simulink model "Vataleni_PMSG_SSO_Final"  (R2025b)
settings: Solver=ode4  StartTime=0.0  StopTime=12  FixedStep=0.00020000000000000001  RelTol=1e-3
model workspace (MAT data in the model file):
  grid_disturbance_time = 2
  mitigation_enable = 0
  scr_final = 10
  scr_initial = 10
  wind_nom = 12
  wind_step = 12
  wind_step_time = 4
settings Model: Creator=Tsenaye  LastModifiedBy=Tsenaye
settings DataIOCC: SignalLogging=off
settings DebuggingCC: AlgebraicLoopMsg=error  UnconnectedInputMsg=error  UnconnectedOutputMsg=warning  UnconnectedLineMsg=error

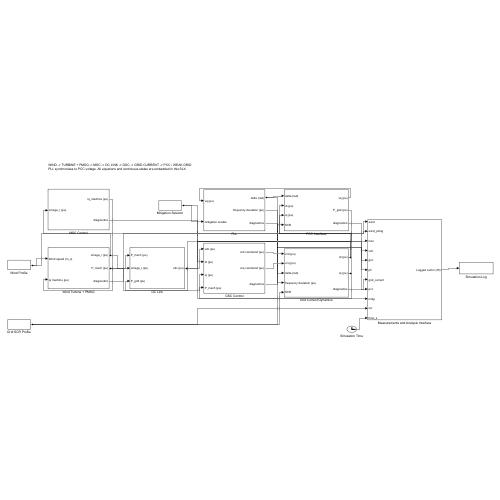
[thumbnail: Simulink's stored preview of the top-level diagram]
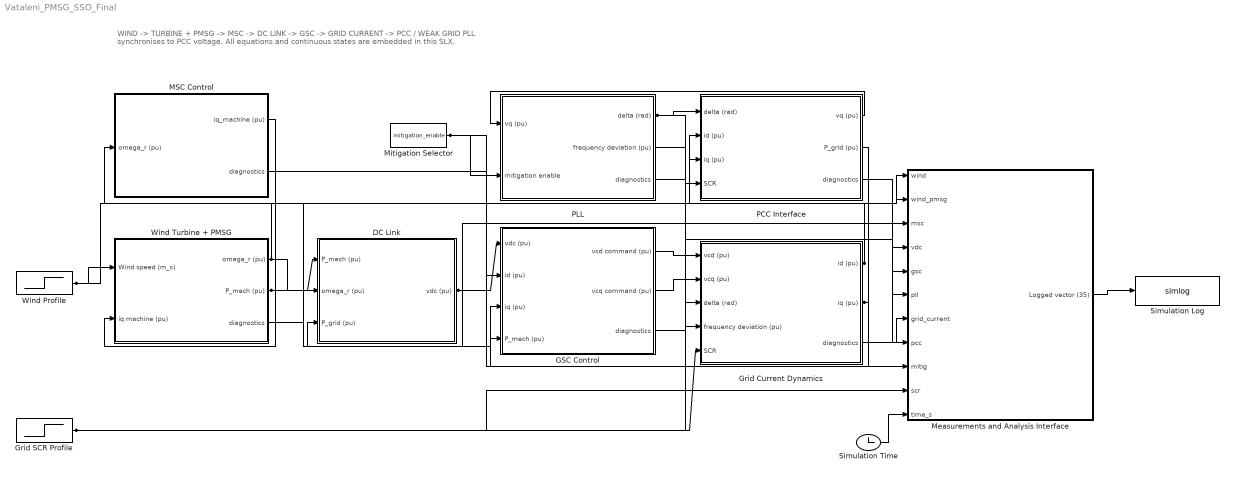
== system Vataleni_PMSG_SSO_Final ==
  note: WIND -> TURBINE + PMSG -> MSC -> DC LINK -> GSC -> GRID CURRENT -> PCC / WEAK GRID
      | PLL synchronises to PCC voltage. All equations and continuous states are embedded in this SLX.
  DC Link : Subsystem
  GSC Control : Subsystem
  Grid Current Dynamics : Subsystem
  Grid SCR Profile : Step  Time=grid_disturbance_time  Before=scr_initial  After=scr_final  SampleTime=0
  MSC Control : Subsystem
  Measurements and Analysis Interface : Subsystem
  Mitigation Selector : Constant  Value=mitigation_enable
  PCC Interface : Subsystem
  PLL : Subsystem
  Simulation Log : ToWorkspace  VariableName=simlog  SampleTime=-1
  Simulation Time : Clock
  Wind Profile : Step  Time=wind_step_time  Before=wind_nom  After=wind_step  SampleTime=0
  Wind Turbine + PMSG : Subsystem
  wires:
  Wind Profile/1 -> Wind Turbine + PMSG/1(Wind speed (m_s)), Measurements and Analysis Interface/1(wind)
  MSC Control/1(iq_machine (pu)) -> Wind Turbine + PMSG/2(iq machine (pu))
  Wind Turbine + PMSG/1(omega_r (pu)) -> MSC Control/1(omega_r (pu)), DC Link/2(omega_r (pu))
  Wind Turbine + PMSG/2(P_mech (pu)) -> DC Link/1(P_mech (pu)), GSC Control/4(P_mech (pu))
  PCC Interface/2(P_grid (pu)) -> DC Link/3(P_grid (pu))
  DC Link/1(vdc (pu)) -> GSC Control/1(vdc (pu)), Measurements and Analysis Interface/4(vdc)
  Grid Current Dynamics/1(id (pu)) -> GSC Control/2(id (pu)), PCC Interface/2(id (pu))
  Grid Current Dynamics/2(iq (pu)) -> GSC Control/3(iq (pu)), PCC Interface/3(iq (pu))
  PCC Interface/1(vq (pu)) -> PLL/1(vq (pu))
  Mitigation Selector/1 -> PLL/2(mitigation enable), Measurements and Analysis Interface/9(mitig)
  GSC Control/1(vcd command (pu)) -> Grid Current Dynamics/1(vcd (pu))
  GSC Control/2(vcq command (pu)) -> Grid Current Dynamics/2(vcq (pu))
  PLL/1(delta (rad)) -> Grid Current Dynamics/3(delta (rad)), PCC Interface/1(delta (rad))
  PLL/2(frequency deviation (pu)) -> Grid Current Dynamics/4(frequency deviation (pu))
  Grid SCR Profile/1 -> Grid Current Dynamics/5(SCR), PCC Interface/4(SCR), Measurements and Analysis Interface/10(scr)
  Wind Turbine + PMSG/3(diagnostics) -> Measurements and Analysis Interface/2(wind_pmsg)
  MSC Control/2(diagnostics) -> Measurements and Analysis Interface/3(msc)
  GSC Control/3(diagnostics) -> Measurements and Analysis Interface/5(gsc)
  PLL/3(diagnostics) -> Measurements and Analysis Interface/6(pll)
  Grid Current Dynamics/3(diagnostics) -> Measurements and Analysis Interface/7(grid_current)
  PCC Interface/3(diagnostics) -> Measurements and Analysis Interface/8(pcc)
  Simulation Time/1 -> Measurements and Analysis Interface/11(time_s)
  Measurements and Analysis Interface/1(Logged vector (35)) -> Simulation Log/1

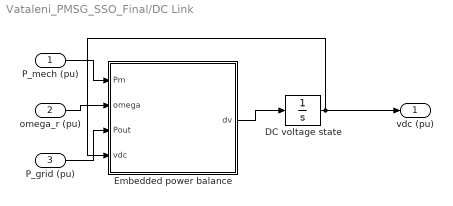
== system Vataleni_PMSG_SSO_Final/DC Link ==
  P_mech (pu) : Inport
  omega_r (pu) : Inport  Port=2
  P_grid (pu) : Inport  Port=3
  DC voltage state : Integrator  InitialCondition=1
  Embedded power balance : MATLAB Function  TreatAsAtomicUnit=on
  vdc (pu) : Outport
  wires:
  P_mech (pu)/1 -> Embedded power balance/1(Pm)
  omega_r (pu)/1 -> Embedded power balance/2(omega)
  P_grid (pu)/1 -> Embedded power balance/3(Pout)
  DC voltage state/1 -> Embedded power balance/4(vdc), vdc (pu)/1
  Embedded power balance/1(dv) -> DC voltage state/1

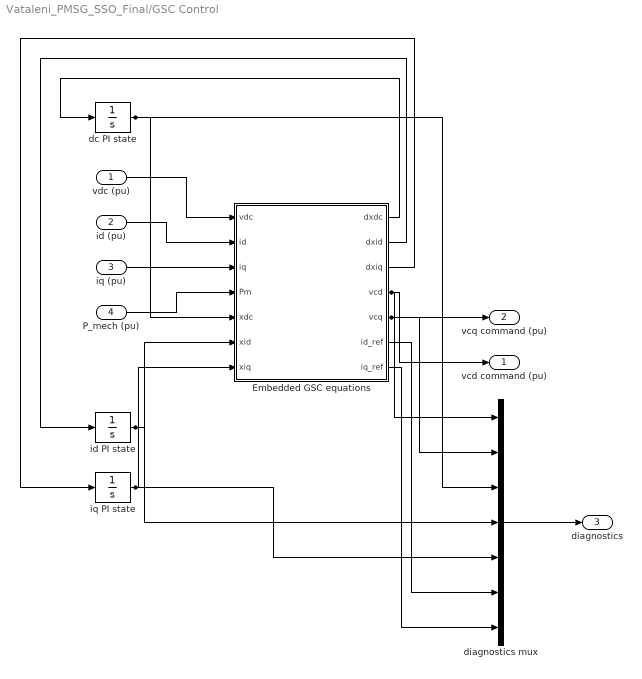
== system Vataleni_PMSG_SSO_Final/GSC Control ==
  vdc (pu) : Inport
  id (pu) : Inport  Port=2
  iq (pu) : Inport  Port=3
  P_mech (pu) : Inport  Port=4
  Embedded GSC equations : MATLAB Function  TreatAsAtomicUnit=on
  dc PI state : Integrator  InitialCondition=-0.0043132729709667306
  diagnostics mux : Mux  Inputs=7
  id PI state : Integrator  InitialCondition=0.013689040731538427
  iq PI state : Integrator
  vcd command (pu) : Outport
  vcq command (pu) : Outport  Port=2
  diagnostics : Outport  Port=3
  wires:
  vdc (pu)/1 -> Embedded GSC equations/1(vdc)
  iq PI state/1 -> diagnostics mux/5, Embedded GSC equations/7(xiq)
  Embedded GSC equations/1(dxdc) -> dc PI state/1
  id PI state/1 -> diagnostics mux/4, Embedded GSC equations/6(xid)
  dc PI state/1 -> diagnostics mux/3, Embedded GSC equations/5(xdc)
  P_mech (pu)/1 -> Embedded GSC equations/4(Pm)
  iq (pu)/1 -> Embedded GSC equations/3(iq)
  id (pu)/1 -> Embedded GSC equations/2(id)
  Embedded GSC equations/2(dxid) -> id PI state/1
  Embedded GSC equations/3(dxiq) -> iq PI state/1
  Embedded GSC equations/4(vcd) -> vcd command (pu)/1, diagnostics mux/1
  Embedded GSC equations/5(vcq) -> vcq command (pu)/1, diagnostics mux/2
  Embedded GSC equations/6(id_ref) -> diagnostics mux/6
  Embedded GSC equations/7(iq_ref) -> diagnostics mux/7
  diagnostics mux/1 -> diagnostics/1

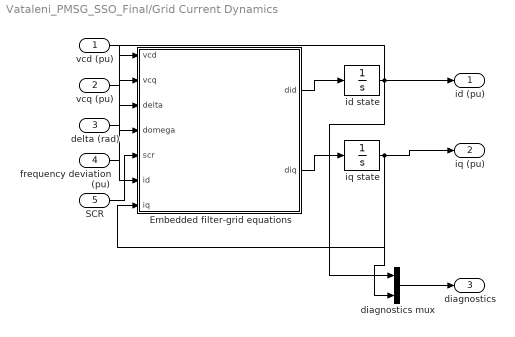
== system Vataleni_PMSG_SSO_Final/Grid Current Dynamics ==
  vcd (pu) : Inport
  vcq (pu) : Inport  Port=2
  delta (rad) : Inport  Port=3
  frequency deviation (pu) : Inport  Port=4
  SCR : Inport  Port=5
  Embedded filter-grid equations : MATLAB Function  TreatAsAtomicUnit=on
  diagnostics mux : Mux  Inputs=2
  id state : Integrator  InitialCondition=0.8771883675516966
  iq state : Integrator
  id (pu) : Outport
  iq (pu) : Outport  Port=2
  diagnostics : Outport  Port=3
  wires:
  vcd (pu)/1 -> Embedded filter-grid equations/1(vcd)
  vcq (pu)/1 -> Embedded filter-grid equations/2(vcq)
  delta (rad)/1 -> Embedded filter-grid equations/3(delta)
  frequency deviation (pu)/1 -> Embedded filter-grid equations/4(domega)
  SCR/1 -> Embedded filter-grid equations/5(scr)
  id state/1 -> Embedded filter-grid equations/6(id), id (pu)/1, diagnostics mux/1
  iq state/1 -> Embedded filter-grid equations/7(iq), iq (pu)/1, diagnostics mux/2
  Embedded filter-grid equations/1(did) -> id state/1
  Embedded filter-grid equations/2(diq) -> iq state/1
  diagnostics mux/1 -> diagnostics/1

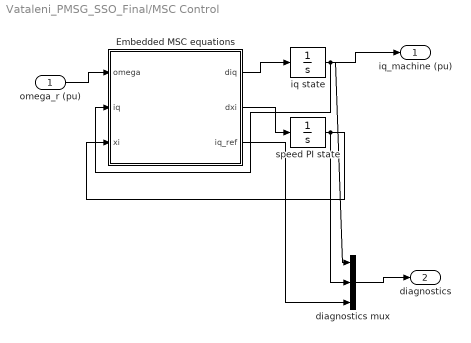
== system Vataleni_PMSG_SSO_Final/MSC Control ==
  omega_r (pu) : Inport
  Embedded MSC equations : MATLAB Function  TreatAsAtomicUnit=on
  diagnostics mux : Mux  Inputs=3
  iq state : Integrator  InitialCondition=0.88150164052266333
  speed PI state : Integrator  InitialCondition=0.88150164052266333
  iq_machine (pu) : Outport
  diagnostics : Outport  Port=2
  wires:
  omega_r (pu)/1 -> Embedded MSC equations/1(omega)
  iq state/1 -> Embedded MSC equations/2(iq), iq_machine (pu)/1, diagnostics mux/1
  speed PI state/1 -> Embedded MSC equations/3(xi), diagnostics mux/2
  Embedded MSC equations/1(diq) -> iq state/1
  Embedded MSC equations/2(dxi) -> speed PI state/1
  Embedded MSC equations/3(iq_ref) -> diagnostics mux/3
  diagnostics mux/1 -> diagnostics/1

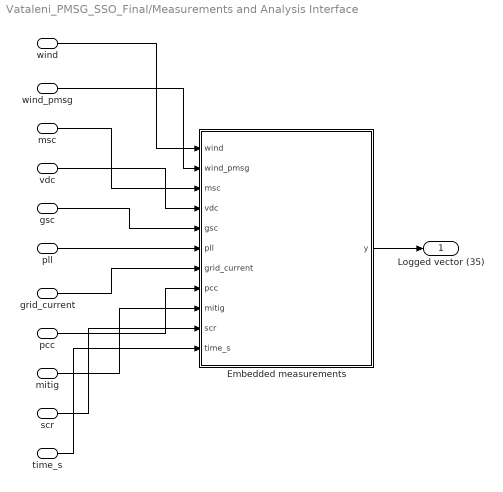
== system Vataleni_PMSG_SSO_Final/Measurements and Analysis Interface ==
  wind : Inport
  wind_pmsg : Inport  Port=2
  msc : Inport  Port=3
  vdc : Inport  Port=4
  gsc : Inport  Port=5
  pll : Inport  Port=6
  grid_current : Inport  Port=7
  pcc : Inport  Port=8
  mitig : Inport  Port=9
  scr : Inport  Port=10
  time_s : Inport  Port=11
  Embedded measurements : MATLAB Function  TreatAsAtomicUnit=on
  Logged vector (35) : Outport
  wires:
  grid_current/1 -> Embedded measurements/7(grid_current)
  gsc/1 -> Embedded measurements/5(gsc)
  time_s/1 -> Embedded measurements/11(time_s)
  msc/1 -> Embedded measurements/3(msc)
  wind/1 -> Embedded measurements/1(wind)
  pcc/1 -> Embedded measurements/8(pcc)
  Embedded measurements/1(y) -> Logged vector (35)/1
  pll/1 -> Embedded measurements/6(pll)
  vdc/1 -> Embedded measurements/4(vdc)
  scr/1 -> Embedded measurements/10(scr)
  wind_pmsg/1 -> Embedded measurements/2(wind_pmsg)
  mitig/1 -> Embedded measurements/9(mitig)

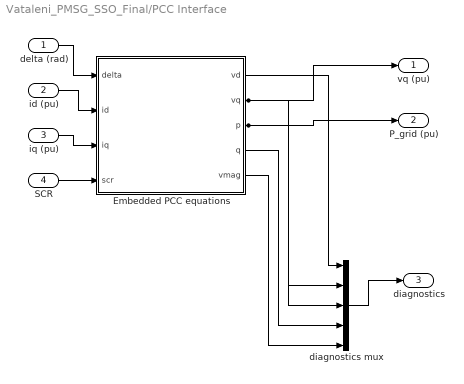
== system Vataleni_PMSG_SSO_Final/PCC Interface ==
  delta (rad) : Inport
  id (pu) : Inport  Port=2
  iq (pu) : Inport  Port=3
  SCR : Inport  Port=4
  Embedded PCC equations : MATLAB Function  TreatAsAtomicUnit=on
  diagnostics mux : Mux  Inputs=5
  vq (pu) : Outport
  P_grid (pu) : Outport  Port=2
  diagnostics : Outport  Port=3
  wires:
  delta (rad)/1 -> Embedded PCC equations/1(delta)
  id (pu)/1 -> Embedded PCC equations/2(id)
  iq (pu)/1 -> Embedded PCC equations/3(iq)
  SCR/1 -> Embedded PCC equations/4(scr)
  Embedded PCC equations/2(vq) -> vq (pu)/1, diagnostics mux/2
  Embedded PCC equations/3(p) -> P_grid (pu)/1, diagnostics mux/3
  Embedded PCC equations/1(vd) -> diagnostics mux/1
  Embedded PCC equations/4(q) -> diagnostics mux/4
  Embedded PCC equations/5(vmag) -> diagnostics mux/5
  diagnostics mux/1 -> diagnostics/1

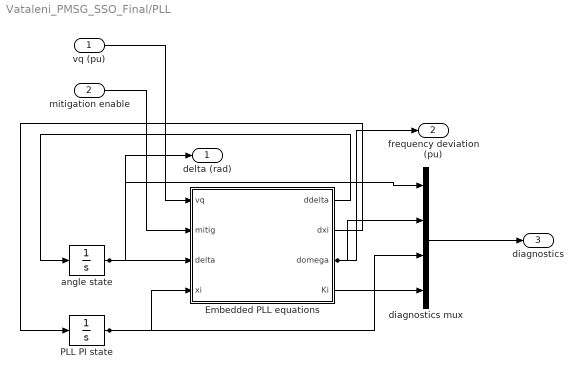
== system Vataleni_PMSG_SSO_Final/PLL ==
  vq (pu) : Inport
  mitigation enable : Inport  Port=2
  Embedded PLL equations : MATLAB Function  TreatAsAtomicUnit=on
  PLL PI state : Integrator
  angle state : Integrator  InitialCondition=0.087831721542046673
  diagnostics mux : Mux
  delta (rad) : Outport
  frequency deviation (pu) : Outport  Port=2
  diagnostics : Outport  Port=3
  wires:
  PLL PI state/1 -> diagnostics mux/3, Embedded PLL equations/4(xi)
  Embedded PLL equations/1(ddelta) -> angle state/1
  angle state/1 -> delta (rad)/1, Embedded PLL equations/3(delta), diagnostics mux/1
  mitigation enable/1 -> Embedded PLL equations/2(mitig)
  vq (pu)/1 -> Embedded PLL equations/1(vq)
  Embedded PLL equations/4(Ki) -> diagnostics mux/4
  Embedded PLL equations/3(domega) -> frequency deviation (pu)/1, diagnostics mux/2
  Embedded PLL equations/2(dxi) -> PLL PI state/1
  diagnostics mux/1 -> diagnostics/1

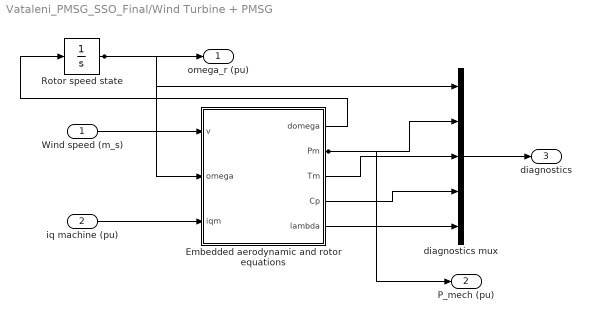
== system Vataleni_PMSG_SSO_Final/Wind Turbine + PMSG ==
  Wind speed (m_s) : Inport
  iq machine (pu) : Inport  Port=2
  Embedded aerodynamic and rotor equations : MATLAB Function  TreatAsAtomicUnit=on
  Rotor speed state : Integrator  InitialCondition=1
  diagnostics mux : Mux  Inputs=5
  omega_r (pu) : Outport
  P_mech (pu) : Outport  Port=2
  diagnostics : Outport  Port=3
  wires:
  Rotor speed state/1 -> diagnostics mux/1, omega_r (pu)/1, Embedded aerodynamic and rotor equations/2(omega)
  iq machine (pu)/1 -> Embedded aerodynamic and rotor equations/3(iqm)
  Wind speed (m_s)/1 -> Embedded aerodynamic and rotor equations/1(v)
  Embedded aerodynamic and rotor equations/1(domega) -> Rotor speed state/1
  Embedded aerodynamic and rotor equations/3(Tm) -> diagnostics mux/3
  Embedded aerodynamic and rotor equations/2(Pm) -> P_mech (pu)/1, diagnostics mux/2
  Embedded aerodynamic and rotor equations/5(lambda) -> diagnostics mux/5
  Embedded aerodynamic and rotor equations/4(Cp) -> diagnostics mux/4
  diagnostics mux/1 -> diagnostics/1

== matlab function Vataleni_PMSG_SSO_Final/Measurements and Analysis Interface/Embedded measurements ==
  data: wind input; y output; wind_pmsg input; msc input; vdc input; gsc input; pll input; grid_current input; pcc input; mitig input; scr input; time_s input
function y = measurements(wind,wind_pmsg,msc,vdc,gsc,pll,grid_current,pcc,mitig,scr,time_s)
%#codegen
omega=wind_pmsg(1); Pm=wind_pmsg(2); Tm=wind_pmsg(3); Cp=wind_pmsg(4); lambda=wind_pmsg(5);
iqm=msc(1); xi_m=msc(2); iqm_ref=msc(3);
vcd=gsc(1); vcq=gsc(2); xi_dc=gsc(3); xi_id=gsc(4); xi_iq=gsc(5); id_ref=gsc(6); iq_ref=gsc(7);
delta=pll(1); domega=pll(2); xi_pll=pll(3); pll_ki=pll(4);
id=grid_current(1); iq=grid_current(2);
vd=pcc(1); vq=pcc(2); p=pcc(3); q=pcc(4); vmag=pcc(5);
theta=314.15926535897933*time_s+delta; Ibase=4183.6976028233748; Vphase=398.37168574084183;
ia=sqrt(2)*Ibase*(id*cos(theta)-iq*sin(theta)); va=sqrt(2)*Vphase*(vd*cos(theta)-vq*sin(theta));
imag=hypot(id,iq); Ki=pll_ki;
y=[wind;omega;Tm;Pm;iqm;vdc;id;iq;p;q;vd;vq;vmag;delta;ia;va;imag;scr;Cp;lambda; ...
omega;omega;iqm;0;iqm_ref;vcd;vcq;50*(1+domega);p;Ki;domega;1;id_ref;iq_ref;pll_ki];
xi_m=xi_m; xi_dc=xi_dc; xi_id=xi_id; xi_iq=xi_iq; xi_pll=xi_pll;
end

== matlab function Vataleni_PMSG_SSO_Final/MSC Control/Embedded MSC equations ==
  data: omega input; diq output; iq input; xi input; dxi output; iq_ref output
function [diq,dxi,iq_ref] = control(omega,iq,xi)
%#codegen
iq_ref=2*(omega-1)+xi; diq=(iq_ref-iq)/0.02; dxi=1*(omega-1);
end

== matlab function Vataleni_PMSG_SSO_Final/Wind Turbine + PMSG/Embedded aerodynamic and rotor equations ==
  data: v input; domega output; omega input; iqm input; Pm output; Tm output; Cp output; lambda output
function [domega,Pm,Tm,Cp,lambda] = dynamics(v,omega,iqm)
%#codegen
v=max(double(v),0.1); omega=max(double(omega),0.05);
lambda=(omega*1.3745454545454545)*55/v; beta=0;
invli=1/(lambda+0.08*beta)-0.035/(beta^3+1); li=1/max(invli,1e-3);
Cp=0.22*(116/li-0.4*beta-5)*exp(-12.5/li); Cp=min(max(Cp,0),0.50);
Pwind=0.5*1.2250000000000001*9503.317777109125*Cp*v^3; Pm=min(max(Pwind/5000000,0),1.15);
Tm=Pm/omega; domega=(Tm-iqm-0.02*(omega-1))/(2*4);
end

== matlab function Vataleni_PMSG_SSO_Final/DC Link/Embedded power balance ==
  data: Pm input; dv output; omega input; Pout input; vdc input
function dv = dynamics(Pm,omega,Pout,vdc)
%#codegen
dv=(Pm*omega-Pout)/(0.080000000000000002*max(vdc,0.25));
end

== matlab function Vataleni_PMSG_SSO_Final/GSC Control/Embedded GSC equations ==
  data: vdc input; dxdc output; id input; iq input; Pm input; xdc input; xid input; xiq input; dxid output; dxiq output; vcd output; vcq output; id_ref output; iq_ref output
function [dxdc,dxid,dxiq,vcd,vcq,id_ref,iq_ref] = control(vdc,id,iq,Pm,xdc,xid,xiq)
%#codegen
id_ref=Pm+0.80000000000000004*(vdc-1)+xdc; iq_ref=0;
vcd=1+0.29999999999999999*(id_ref-id)+xid-0.14999999999999999*iq;
vcq=0.29999999999999999*(iq_ref-iq)+xiq+0.14999999999999999*id;
dxdc=20*(vdc-1); dxid=20*(id_ref-id); dxiq=20*(iq_ref-iq);
end

== matlab function Vataleni_PMSG_SSO_Final/PLL/Embedded PLL equations ==
  data: vq input; ddelta output; mitig input; delta input; xi input; dxi output; domega output; Ki output
function [ddelta,dxi,domega,Ki] = control(vq,mitig,delta,xi)
%#codegen
if mitig>0.5, Ki=0.5; else, Ki=2.7999999999999998; end
domega=0.01*vq+xi; dxi=Ki*vq; ddelta=314.15926535897933*domega; delta=delta;
end

== matlab function Vataleni_PMSG_SSO_Final/Grid Current Dynamics/Embedded filter-grid equations ==
  data: vcd input; did output; vcq input; delta input; domega input; scr input; id input; iq input; diq output
function [did,diq] = dynamics(vcd,vcq,delta,domega,scr,id,iq)
%#codegen
Xg=1/max(scr,0.1); Rg=Xg/10; Lt=0.14999999999999999+Xg; R=0.01+Rg; E=1;
did=314.15926535897933/Lt*(vcd-E*cos(delta)-R*id+Lt*(1+domega)*iq);
diq=314.15926535897933/Lt*(vcq+E*sin(delta)-R*iq-Lt*(1+domega)*id);
end

== matlab function Vataleni_PMSG_SSO_Final/PCC Interface/Embedded PCC equations ==
  data: delta input; vd output; id input; iq input; scr input; vq output; p output; q output; vmag output
function [vd,vq,p,q,vmag] = interface(delta,id,iq,scr)
%#codegen
Xg=1/max(scr,0.1); Rg=Xg/10; E=1;
vd=E*cos(delta)+Rg*id-Xg*iq; vq=-E*sin(delta)+Rg*iq+Xg*id;
p=vd*id+vq*iq; q=vq*id-vd*iq; vmag=hypot(vd,vq);
end
